simulink model "DAB_RA8P1_Final_Physical_MOSFET"  (R2024b)
settings: Solver=daessc  StartTime=0.0  StopTime=0.03  MaxStep=1e-8  RelTol=2e-3  AbsTol=1e-5
libraries: ee_lib x118, fl_lib x18, nesl_utility x15
(part 6 of 6)

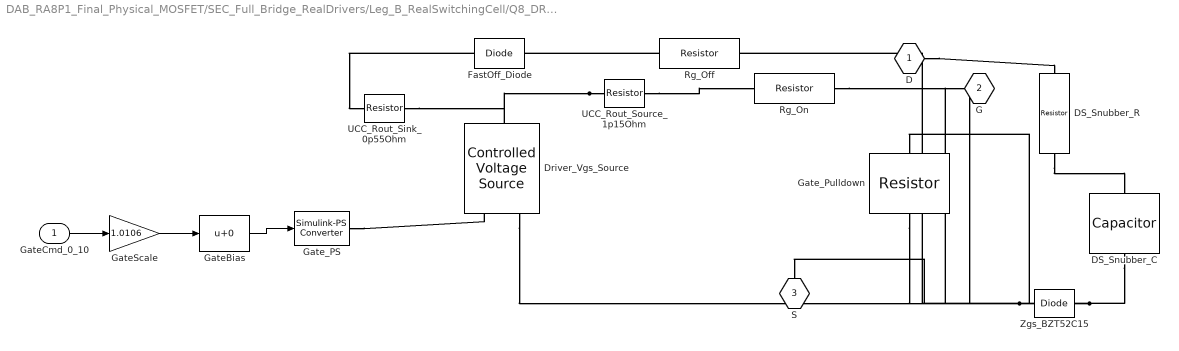
== system DAB_RA8P1_Final_Physical_MOSFET/SEC_Full_Bridge_RealDrivers/Leg_B_RealSwitchingCell/Q8_DRV_EQ ==
  GateCmd_0_10 : Inport
  DS_Snubber_C : ee_lib/Passive/Capacitor  cap_option=ee.enum.passive.capacitor.capOption.const  c=470 pF  Cvec=[1e-05, 1e-06] F  Vvec=[0, 10] V  CV_table_symmetry=ee.enum.passive.capacitor.tableSymmetry.yes  f_vec=[1, 10] kHz  DFext_vec=[.8, 1.2]  enable_C_tol=ee.enum.toleranceApplication.none  averaging_period=0 s  C_tol=5  tol_distribution=ee.enum.toleranceDistribution.uniform  nSigma=4  r=0.05 Ohm  g=0 1/Ohm  enable_operating_limits=ee.enum.enable.no  operating_limit_action=ee.enum.passive.reportOpLim.warn  max_working_voltage_range=[-25, 25] V  power_rating=1 W  maxTemperature=85 degC  thermalEnable=false  thermalMass=1 J/K  fault_action=simscape.enum.assert.action.none  t_fault=1 s  i_specify=off  i_priority=None  i=0 A  i_nominal_specify=off  i_nominal_value=1  i_nominal_unit=A  v_specify=off  v_priority=None  v=0 V  v_nominal_specify=off  v_nominal_value=1  v_nominal_unit=V  vc_specify=off  vc_priority=High  vc=0 V  vc_nominal_specify=off  vc_nominal_value=1  vc_nominal_unit=V  T_specify=off  T_priority=None  T=298.15 K  T_nominal_specify=off  T_nominal_value=1  T_nominal_unit=K
      settings: AttributesFormatString=Initial 470pF C0G snubber; DNP/tune after Vds measurement
  DS_Snubber_R : ee_lib/Passive/Resistor  R=10 Ohm  enable_R_tol=ee.enum.toleranceApplication.none  R_tol=5  tol_distribution=ee.enum.toleranceDistribution.uniform  nSigma=4  enable_operating_limits=ee.enum.enable.no  operating_limit_action=ee.enum.passive.reportOpLim.warn  power_rating=1 W  max_working_voltage=100 V  noise_mode=ee.enum.sources.noise.Disabled  Tdevice=25 degC  sample_time=1e-3 s  repeatability=ee.enum.ic.repeatability.notRepeatable  user_seed=0  auto_seed=1141249012  fault_action=simscape.enum.assert.action.none  t_fault=1 s  power_derating_T1=70 degC  power_derating_T2=155 degC  operating_temperature_range_vec=[-50, 150] degC  alpha=3.93e-3 1/K  Tmeas=25 degC  thermal_mass=100 J/K  temperature_specify=off  temperature_priority=High  temperature=298.15 K  temperature_nominal_specify=off  temperature_nominal_value=1  temperature_nominal_unit=K
      settings: AttributesFormatString=Initial RC snubber value; tune by double-pulse measurement
  Driver_Vgs_Source : fl_lib/Electrical/Electrical Sources/Controlled Voltage Source
  FastOff_Diode : ee_lib/Semiconductors & Converters/Diode  ModelType=ee.enum.diode.modelType.pwl  TableType=ee.enum.diode.tableType.IfMat  IfMat=[.07, .12, .19, 1.75, 4.24, 7.32, 11.2; .16, .3, .72, 2.14, 5.02, 8.35, 13.12] A  VfMat=[.9, 1.15, 1.25, 1.5, 1.75, 2.17, 2.6, 2.85; .58, .68, .75, 1.1, 1.38, 1.77, 2.27, 2.7] V  TjVec=[25, 125] degC  VfVec=[.5, .7, .9, 1.3, 1.7, 2.1, 2.5] V  IfVec=[.1, .2, .5, 1, 2, 4, 7, 10] A  IrMat=[1e-06, 2e-06, 5e-06, 1e-05, 2.5e-05, 5e-05, .0001; 2e-06, 5e-06, 1e-05, 4e-05, 8e-05, .0002, .0005] A  VrMat=[10, 100, 200, 250, 300, 325, 350; 10, 70, 160, 220, 270, 300, 320] V  VrVec=[10, 20, 40, 50, 70, 80, 100] V  IrVec=[1e-06, 2e-06, 5e-06, 1e-05, 2e-05, 5e-05, .0001] A  Vf=0.30 V  Ron=0.19 Ohm  Goff=1e-8 S  prmExp=ee.enum.diode.expParam.useTwo  I12=[.0137, .545] A  V12=[.6, .7] V  RS=0 Ohm  Tmeas=298.15 K  IS=1e-12 A  ec=1  I1=0.0137 A  V1=0.6 V  N_series=1  N_parallel=1  ZenerEnable=false  Rz=0.3 Ohm  BV=40 V  C_param=ee.enum.diode.capParam.fixed  CJ=0 pF  CJ0=5 pF  Vvec=[.1, 10, 100] V  Cvec=[3.5, 1, .4] pF  VJ=1 V  Mgrad=0.5  FC=0.5  Q_param=ee.enum.diode.recoveryParam.off  iRM=-7.15 A  iF=4 A  didt=-750 A/us  trr_factor=3  trr=115 ns  Qrr=150 nA*s  Vr=-600 V  Ls=150 nH  Erec=0.03 J  TT=50 ns  tau=100 ns  T_param=ee.enum.diode.temperatureParam.off  Tdevice=298.15 K  I1_T2=0.245 A  V1_T2=0.5 V  IS_T2=1.25e-7 A  Tmeas2=125 degC  XTI_param=ee.enum.diode.xtiParam.pn  XTI=3  EG_param=ee.enum.diode.egapParam.material_si  EG=1.11 eV  dBVdT=0 V/K  fault_action=simscape.enum.assert.action.none  t_fault=inf s  enable_fault_input=simscape.enum.onoff.off  i_specify=off  i_priority=None  i=0 A  i_nominal_specify=off  i_nominal_value=1  i_nominal_unit=A  v_specify=off  v_priority=None  v=0 V  v_nominal_specify=off  v_nominal_value=1  v_nominal_unit=V  v_capacitor_specify=off  v_capacitor_priority=None  v_capacitor=0 V  v_capacitor_nominal_specify=off  v_capacitor_nominal_value=1  v_capacitor_nominal_unit=V  Qj_specify=off  Qj_priority=High  Qj=0 C  Qj_nominal_specify=off  Qj_nominal_value=1  Qj_nominal_unit=C  i_diode_specify=off  i_diode_priority=None  i_diode=0 A  i_diode_nominal_specify=off  i_diode_nominal_value=1  i_diode_nominal_unit=A  v_diode_specify=off  v_diode_priority=None  v_diode=0 V  v_diode_nominal_specify=off  v_diode_nominal_value=1  v_diode_nominal_unit=V  i_capacitor_specify=off  i_capacitor_priority=None  i_capacitor=0 A  i_capacitor_nominal_specify=off  i_capacitor_nominal_value=1  i_capacitor_nominal_unit=A  power_dissipated_specify=off  power_dissipated_priority=None  power_dissipated=0 W  power_dissipated_nominal_specify=off  power_dissipated_nominal_value=1  power_dissipated_nominal_unit=W  fidelity_level=ee.enum.diode.fidelity.includeChargeDyn  rec_loss_model=ee.enum.diode.reverseRecoveryModel.fixed  ErecVal=0 J  scaleWithIandV=true  ErecMat=zeros(2, 3) J  TjrecVec=[298.15, 398.15] K  IfrecVec=[.1, 1, 10] A  IrecVal=10 A  VrecVal=10 V  tFilter=1 / 1000 / 100 s  thermal_network_parameterization=ee.enum.thermalNetworkTopology.junctionCase  Rth=[0, 10] K/W  Rth_Cauer=[1, 3, 10] K/W  Rth_Foster=[.08, .14, .22, .16] K/W  thermal_mass_parameterization=ee.enum.thermalNetwork.timeconstant  thermal_mass=[0, 1] J/K  thermal_mass_Cauer=[.1, .3, 1] J/K  thermal_mass_Foster=[.001, .005, .05, .5] J/K  thermal_time_constant=[0, 10] s  thermal_time_constant_Cauer=[1, 3, 10] s  thermal_time_constant_Foster=[7e-05, .0007, .01, .08] s  thermal_mass_initial_temperatures=[25, 25] degC  thermal_mass_initial_temperatures_Cauer=[25, 25, 25] degC  junction_thermal_mass=0.01 J/K  Tvec_initial_Foster=[25, 25, 25, 25] degC  no_thermal_network=0  junction_temperature_specify=off  junction_temperature_priority=None  junction_temperature=25 degC  junction_temperature_nominal_specify=off  junction_temperature_nominal_value=1  junction_temperature_nominal_unit=degC
  GateBias : Bias  SaturateOnIntegerOverflow=off
  GateScale : Gain  Gain=1.0106
  Gate_PS : nesl_utility/Simulink-PS Converter  PhysicalDomain=network_engine_domain  SubClassName=ps_input  LeftPortType=input  RightPortType=output  PseudoPeriodic=off  Frequencies=[]  NoiseDistribution=none  NoiseParameters=[]  Unit=V  AffineConversion=off  FilteringAndDerivatives=provide  SimscapeFilterOrder=1  InputFilterTimeConstant=0.001  UdotUserProvided=0
  Gate_Pulldown : ee_lib/Passive/Resistor  R=10000 Ohm  enable_R_tol=ee.enum.toleranceApplication.none  R_tol=5  tol_distribution=ee.enum.toleranceDistribution.uniform  nSigma=4  enable_operating_limits=ee.enum.enable.no  operating_limit_action=ee.enum.passive.reportOpLim.warn  power_rating=1 W  max_working_voltage=100 V  noise_mode=ee.enum.sources.noise.Disabled  Tdevice=25 degC  sample_time=1e-3 s  repeatability=ee.enum.ic.repeatability.notRepeatable  user_seed=0  auto_seed=1157818018  fault_action=simscape.enum.assert.action.none  t_fault=1 s  power_derating_T1=70 degC  power_derating_T2=155 degC  operating_temperature_range_vec=[-50, 150] degC  alpha=3.93e-3 1/K  Tmeas=25 degC  thermal_mass=100 J/K  temperature_specify=off  temperature_priority=High  temperature=298.15 K  temperature_nominal_specify=off  temperature_nominal_value=1  temperature_nominal_unit=K
  Rg_Off : ee_lib/Passive/Resistor  R=2.2 Ohm  enable_R_tol=ee.enum.toleranceApplication.none  R_tol=5  tol_distribution=ee.enum.toleranceDistribution.uniform  nSigma=4  enable_operating_limits=ee.enum.enable.no  operating_limit_action=ee.enum.passive.reportOpLim.warn  power_rating=1 W  max_working_voltage=100 V  noise_mode=ee.enum.sources.noise.Disabled  Tdevice=25 degC  sample_time=1e-3 s  repeatability=ee.enum.ic.repeatability.notRepeatable  user_seed=0  auto_seed=4137157194  fault_action=simscape.enum.assert.action.none  t_fault=1 s  power_derating_T1=70 degC  power_derating_T2=155 degC  operating_temperature_range_vec=[-50, 150] degC  alpha=3.93e-3 1/K  Tmeas=25 degC  thermal_mass=100 J/K  temperature_specify=off  temperature_priority=High  temperature=298.15 K  temperature_nominal_specify=off  temperature_nominal_value=1  temperature_nominal_unit=K
  Rg_On : ee_lib/Passive/Resistor  R=4.7 Ohm  enable_R_tol=ee.enum.toleranceApplication.none  R_tol=5  tol_distribution=ee.enum.toleranceDistribution.uniform  nSigma=4  enable_operating_limits=ee.enum.enable.no  operating_limit_action=ee.enum.passive.reportOpLim.warn  power_rating=1 W  max_working_voltage=100 V  noise_mode=ee.enum.sources.noise.Disabled  Tdevice=25 degC  sample_time=1e-3 s  repeatability=ee.enum.ic.repeatability.notRepeatable  user_seed=0  auto_seed=2368526529  fault_action=simscape.enum.assert.action.none  t_fault=1 s  power_derating_T1=70 degC  power_derating_T2=155 degC  operating_temperature_range_vec=[-50, 150] degC  alpha=3.93e-3 1/K  Tmeas=25 degC  thermal_mass=100 J/K  temperature_specify=off  temperature_priority=High  temperature=298.15 K  temperature_nominal_specify=off  temperature_nominal_value=1  temperature_nominal_unit=K
  UCC_Rout_Sink_0p55Ohm : ee_lib/Passive/Resistor  R=0.55 Ohm  enable_R_tol=ee.enum.toleranceApplication.none  R_tol=5  tol_distribution=ee.enum.toleranceDistribution.uniform  nSigma=4  enable_operating_limits=ee.enum.enable.no  operating_limit_action=ee.enum.passive.reportOpLim.warn  power_rating=1 W  max_working_voltage=100 V  noise_mode=ee.enum.sources.noise.Disabled  Tdevice=25 degC  sample_time=1e-3 s  repeatability=ee.enum.ic.repeatability.notRepeatable  user_seed=0  auto_seed=609397185  fault_action=simscape.enum.assert.action.none  t_fault=1 s  power_derating_T1=70 degC  power_derating_T2=155 degC  operating_temperature_range_vec=[-50, 150] degC  alpha=3.93e-3 1/K  Tmeas=25 degC  thermal_mass=100 J/K  temperature_specify=off  temperature_priority=High  temperature=298.15 K  temperature_nominal_specify=off  temperature_nominal_value=1  temperature_nominal_unit=K
  UCC_Rout_Source_1p15Ohm : ee_lib/Passive/Resistor  R=1.15 Ohm  enable_R_tol=ee.enum.toleranceApplication.none  R_tol=5  tol_distribution=ee.enum.toleranceDistribution.uniform  nSigma=4  enable_operating_limits=ee.enum.enable.no  operating_limit_action=ee.enum.passive.reportOpLim.warn  power_rating=1 W  max_working_voltage=100 V  noise_mode=ee.enum.sources.noise.Disabled  Tdevice=25 degC  sample_time=1e-3 s  repeatability=ee.enum.ic.repeatability.notRepeatable  user_seed=0  auto_seed=3437178441  fault_action=simscape.enum.assert.action.none  t_fault=1 s  power_derating_T1=70 degC  power_derating_T2=155 degC  operating_temperature_range_vec=[-50, 150] degC  alpha=3.93e-3 1/K  Tmeas=25 degC  thermal_mass=100 J/K  temperature_specify=off  temperature_priority=High  temperature=298.15 K  temperature_nominal_specify=off  temperature_nominal_value=1  temperature_nominal_unit=K
  Zgs_BZT52C15 : ee_lib/Semiconductors & Converters/Diode  ModelType=ee.enum.diode.modelType.pwl  TableType=ee.enum.diode.tableType.IfMat  IfMat=[.07, .12, .19, 1.75, 4.24, 7.32, 11.2; .16, .3, .72, 2.14, 5.02, 8.35, 13.12] A  VfMat=[.9, 1.15, 1.25, 1.5, 1.75, 2.17, 2.6, 2.85; .58, .68, .75, 1.1, 1.38, 1.77, 2.27, 2.7] V  TjVec=[25, 125] degC  VfVec=[.5, .7, .9, 1.3, 1.7, 2.1, 2.5] V  IfVec=[.1, .2, .5, 1, 2, 4, 7, 10] A  IrMat=[1e-06, 2e-06, 5e-06, 1e-05, 2.5e-05, 5e-05, .0001; 2e-06, 5e-06, 1e-05, 4e-05, 8e-05, .0002, .0005] A  VrMat=[10, 100, 200, 250, 300, 325, 350; 10, 70, 160, 220, 270, 300, 320] V  VrVec=[10, 20, 40, 50, 70, 80, 100] V  IrVec=[1e-06, 2e-06, 5e-06, 1e-05, 2e-05, 5e-05, .0001] A  Vf=0.60 V  Ron=0.30 Ohm  Goff=1e-8 S  prmExp=ee.enum.diode.expParam.useTwo  I12=[.0137, .545] A  V12=[.6, .7] V  RS=0 Ohm  Tmeas=298.15 K  IS=1e-12 A  ec=1  I1=0.0137 A  V1=0.6 V  N_series=1  N_parallel=1  ZenerEnable=true  Rz=1 Ohm  BV=15 V  C_param=ee.enum.diode.capParam.fixed  CJ=0 pF  CJ0=5 pF  Vvec=[.1, 10, 100] V  Cvec=[3.5, 1, .4] pF  VJ=1 V  Mgrad=0.5  FC=0.5  Q_param=ee.enum.diode.recoveryParam.off  iRM=-7.15 A  iF=4 A  didt=-750 A/us  trr_factor=3  trr=115 ns  Qrr=150 nA*s  Vr=-600 V  Ls=150 nH  Erec=0.03 J  TT=50 ns  tau=100 ns  T_param=ee.enum.diode.temperatureParam.off  Tdevice=298.15 K  I1_T2=0.245 A  V1_T2=0.5 V  IS_T2=1.25e-7 A  Tmeas2=125 degC  XTI_param=ee.enum.diode.xtiParam.pn  XTI=3  EG_param=ee.enum.diode.egapParam.material_si  EG=1.11 eV  dBVdT=0 V/K  fault_action=simscape.enum.assert.action.none  t_fault=inf s  enable_fault_input=simscape.enum.onoff.off  i_specify=off  i_priority=None  i=0 A  i_nominal_specify=off  i_nominal_value=1  i_nominal_unit=A  v_specify=off  v_priority=None  v=0 V  v_nominal_specify=off  v_nominal_value=1  v_nominal_unit=V  v_capacitor_specify=off  v_capacitor_priority=None  v_capacitor=0 V  v_capacitor_nominal_specify=off  v_capacitor_nominal_value=1  v_capacitor_nominal_unit=V  Qj_specify=off  Qj_priority=High  Qj=0 C  Qj_nominal_specify=off  Qj_nominal_value=1  Qj_nominal_unit=C  i_diode_specify=off  i_diode_priority=None  i_diode=0 A  i_diode_nominal_specify=off  i_diode_nominal_value=1  i_diode_nominal_unit=A  v_diode_specify=off  v_diode_priority=None  v_diode=0 V  v_diode_nominal_specify=off  v_diode_nominal_value=1  v_diode_nominal_unit=V  i_capacitor_specify=off  i_capacitor_priority=None  i_capacitor=0 A  i_capacitor_nominal_specify=off  i_capacitor_nominal_value=1  i_capacitor_nominal_unit=A  power_dissipated_specify=off  power_dissipated_priority=None  power_dissipated=0 W  power_dissipated_nominal_specify=off  power_dissipated_nominal_value=1  power_dissipated_nominal_unit=W  fidelity_level=ee.enum.diode.fidelity.includeChargeDyn  rec_loss_model=ee.enum.diode.reverseRecoveryModel.fixed  ErecVal=0 J  scaleWithIandV=true  ErecMat=zeros(2, 3) J  TjrecVec=[298.15, 398.15] K  IfrecVec=[.1, 1, 10] A  IrecVal=10 A  VrecVal=10 V  tFilter=1 / 1000 / 100 s  thermal_network_parameterization=ee.enum.thermalNetworkTopology.junctionCase  Rth=[0, 10] K/W  Rth_Cauer=[1, 3, 10] K/W  Rth_Foster=[.08, .14, .22, .16] K/W  thermal_mass_parameterization=ee.enum.thermalNetwork.timeconstant  thermal_mass=[0, 1] J/K  thermal_mass_Cauer=[.1, .3, 1] J/K  thermal_mass_Foster=[.001, .005, .05, .5] J/K  thermal_time_constant=[0, 10] s  thermal_time_constant_Cauer=[1, 3, 10] s  thermal_time_constant_Foster=[7e-05, .0007, .01, .08] s  thermal_mass_initial_temperatures=[25, 25] degC  thermal_mass_initial_temperatures_Cauer=[25, 25, 25] degC  junction_thermal_mass=0.01 J/K  Tvec_initial_Foster=[25, 25, 25, 25] degC  no_thermal_network=0  junction_temperature_specify=off  junction_temperature_priority=None  junction_temperature=25 degC  junction_temperature_nominal_specify=off  junction_temperature_nominal_value=1  junction_temperature_nominal_unit=degC
  D : PMIOPort  Side=Right
  G : PMIOPort  Port=2  Side=Right
  S : PMIOPort  Port=3  Side=Right
  wires:
  GateCmd_0_10/1 -> GateScale/1
  GateScale/1 -> GateBias/1
  GateBias/1 -> Gate_PS/1
  connections:
  Gate_PS/RConn1 -- Driver_Vgs_Source/RConn1
  Rg_On/RConn1 -- Zgs_BZT52C15/RConn1 -- Rg_Off/LConn1 -- G/RConn1 -- Gate_Pulldown/LConn1
  Rg_Off/RConn1 -- FastOff_Diode/LConn1
  Gate_Pulldown/RConn1 -- Driver_Vgs_Source/RConn2 -- Zgs_BZT52C15/LConn1 -- S/RConn1 -- DS_Snubber_C/RConn1
  D/RConn1 -- DS_Snubber_R/LConn1
  DS_Snubber_R/RConn1 -- DS_Snubber_C/LConn1
  UCC_Rout_Source_1p15Ohm/LConn1 -- Driver_Vgs_Source/LConn1 -- UCC_Rout_Sink_0p55Ohm/RConn1
  UCC_Rout_Source_1p15Ohm/RConn1 -- Rg_On/LConn1
  FastOff_Diode/RConn1 -- UCC_Rout_Sink_0p55Ohm/LConn1

== matlab function DAB_RA8P1_Final_Physical_MOSFET/RA8P1_Realtime_Voltage_PI ==
  settings: updateMethod=DISCRETE  sampleTime=1e-8
  data: t input; g1 output; Vout input; VrefCmd input; Vin input; Iout input; Ipri input; Isec input; g2 output; g3 output; g4 output; g5 output; g6 output; g7 output; g8 output; PhaseUs output; RunReq input; RawFaultN input
function [g1,g2,g3,g4,g5,g6,g7,g8,PhaseUs] = f(t,Vout,VrefCmd,Vin,Iout,Ipri,Isec,RunReq,RawFaultN)
%#codegen
% Cold start: alternating primary three-level pulses, secondary gates off.
% NORMAL mode starts only after 20 consecutive voltage-domain samples.
% RawFaultN is the modeled hardware FAULT_LATCH_N signal.
persistent trim prevErr lastTick vFilt vinFilt iFilt permitCount normalEnabled startupEnabled startupCycle startupPulseAllowed startupPolarity normalRamp iPriPeakHold iSecPeakHold startupPulseCmd startupIpriCyclePeak startupIsecCyclePeak epsTrim epsQuantAcc epsPhaseCmd
if isempty(trim)
    trim = 0;
    prevErr = 0;
    lastTick = -1;
    vFilt = 0;
    vinFilt = 24;
    iFilt = 0;
    permitCount = uint16(0);
    normalEnabled = false;
    startupEnabled = false;
    startupCycle = -1;
    startupPulseAllowed = false;
    startupPolarity = false;
    normalRamp = 0;
    iPriPeakHold = 0;
    iSecPeakHold = 0;
    startupPulseCmd = 100e-9;
    startupIpriCyclePeak = 0;
    startupIsecCyclePeak = 0;
    epsTrim = 0;
    epsQuantAcc = 0;
    epsPhaseCmd = 0.30e-6;
end
fs = 300e3;
T = 1/fs;
deadTime = 120e-9;
TsCtrl = 10e-6;
tick = floor(t/TsCtrl);
Vref = min(max(VrefCmd,36),48);
rawVoltageOk = Vin >= 18 && Vin <= 28 && Vout >= -0.5 && Vout < 50;
faultOk = RunReq > 0.5 && RawFaultN > 0.5 && rawVoltageOk;
iPriPeakHold = max(iPriPeakHold,abs(Ipri));
iSecPeakHold = max(iSecPeakHold,abs(Isec));
startupIpriCyclePeak = max(startupIpriCyclePeak,abs(Ipri));
startupIsecCyclePeak = max(startupIsecCyclePeak,abs(Isec));
if tick ~= lastTick
    if lastTick < 0
        vFilt = Vout;
        vinFilt = Vin;
        iFilt = abs(Iout);
    else
        vFilt = vFilt + 0.40*(Vout - vFilt);
        vinFilt = vinFilt + 0.10*(Vin - vinFilt);
        iFilt = iFilt + 0.22*(abs(Iout) - iFilt);
    end
    ratioMismatch = abs(Vout - 2*Vin);
    entryRatioOk = (Vout < 2*Vin && ratioMismatch <= 7.0) || ...
        (Vout >= 2*Vin && ratioMismatch <= 12.5);
    holdRatioOk = (Vout < 2*Vin && ratioMismatch < 10.0) || ...
        (Vout >= 2*Vin && ratioMismatch < 13.5);
    startupOk = faultOk && vinFilt >= 18 && vinFilt <= 28 && ...
        vFilt >= -0.5 && vFilt < 50;
    entryOk = faultOk && vinFilt >= 18 && vinFilt <= 28 && ...
        vFilt >= 36 && vFilt <= 48 && entryRatioOk;
    holdOk = faultOk && vinFilt >= 18 && vinFilt <= 28 && ...
        vFilt >= 36 && vFilt <= 49.0 && holdRatioOk;
    if normalEnabled
        if ~holdOk
            normalEnabled = false;
            startupEnabled = startupOk;
            startupPulseCmd = startup_pulse_width(Vout,Vin);
            startupCycle = -1;
            startupPolarity = false;
            permitCount = uint16(0);
            trim = 0;
            normalRamp = 0;
        end
    else
        if ~startupOk
            startupEnabled = false;
            permitCount = uint16(0);
        elseif entryOk
            startupEnabled = false;
            if permitCount < uint16(20)
                permitCount = permitCount + uint16(1);
            end
        else
            if ~startupEnabled
                startupPulseCmd = startup_pulse_width(Vout,Vin);
                startupCycle = -1;
                startupPolarity = false;
                startupIpriCyclePeak = 0;
                startupIsecCyclePeak = 0;
            end
            startupEnabled = true;
            permitCount = uint16(0);
        end
        if permitCount >= uint16(20)
            normalEnabled = true;
            startupEnabled = false;
            normalRamp = 0;
            trim = 0;
            prevErr = Vref - vFilt;
        end
    end
    if normalEnabled
        normalIpriLow = min(48,36 + 1.2*iFilt);
        normalIsecLow = min(24,18 + 0.6*iFilt);
        if iPriPeakHold < normalIpriLow && iSecPeakHold < normalIsecLow
            normalRamp = min(1,normalRamp + 0.005);
        elseif iPriPeakHold >= normalIpriLow + 4 || iSecPeakHold >= normalIsecLow + 2
            normalRamp = max(0,normalRamp - 0.05);
        end
        err = Vref - vFilt;
        dErr = err - prevErr;
        trim = 0.965*trim + 0.0102e-6*err + 0.0033e-6*dErr;
        trimLimit = 0.100e-6;
        if iFilt < 0.70
            trimLimit = 0.016e-6;
        end
        trim = min(max(trim, -trimLimit), trimLimit);
        prevErr = err;
        if iFilt >= 4
            epsTrim = min(max(epsTrim + 0.5e-9*err,-25e-9),25e-9);
            epsDesired = min(max(0.295e-6 + epsTrim + 0.20e-6*err,0.28e-6),0.32e-6);
            epsLow = floor(epsDesired/10e-9)*10e-9;
            epsQuantAcc = epsQuantAcc + (epsDesired-epsLow)/10e-9;
            epsPhaseCmd = epsLow;
            if epsQuantAcc >= 1
                epsPhaseCmd = epsLow + 10e-9;
                epsQuantAcc = epsQuantAcc - 1;
            end
        else
            epsTrim = 0;
            epsQuantAcc = 0;
            epsPhaseCmd = 0.30e-6;
        end
    else
        trim = 0;
        normalRamp = 0;
        epsTrim = 0;
        epsQuantAcc = 0;
        epsPhaseCmd = 0.30e-6;
    end
    iPriPeakHold = abs(Ipri);
    iSecPeakHold = abs(Isec);
    lastTick = tick;
end
if normalEnabled && faultOk && iFilt >= 4
    % Physical-model EPS PI around the measured 0.295 us balance point.
    % epsPhaseCmd uses 10 ns timer quantization with pulse-density dither.
    if iPriPeakHold < 50 && iSecPeakHold < 28
        inner = 0.20e-6;
        phase = epsPhaseCmd;
        [a,an] = halfbridge(t,T,deadTime);
        [b,bn] = halfbridge(t+T/2-inner,T,deadTime);
        [c,cn] = halfbridge(t-phase,T,deadTime);
        [d,dn] = halfbridge(t-phase+T/2,T,deadTime);
        g1 = 10*a;  g2 = 10*an;
        g3 = 10*b;  g4 = 10*bn;
        g5 = 10*c;  g6 = 10*cn;
        g7 = 10*d;  g8 = 10*dn;
        PhaseUs = phase*1e6;
    else
        g1 = 0; g2 = 0; g3 = 0; g4 = 0;
        g5 = 0; g6 = 0; g7 = 0; g8 = 0;
        PhaseUs = 0;
    end
elseif normalEnabled && faultOk
    phase = normalRamp*(base_phase(Vref, vinFilt, iFilt) + trim);
    phase = min(max(phase, -0.55e-6), 0.46e-6);
    [a,an] = halfbridge(t,T,deadTime);
    [b,bn] = halfbridge(t+T/2,T,deadTime);
    [c,cn] = halfbridge(t-phase,T,deadTime);
    [d,dn] = halfbridge(t-phase+T/2,T,deadTime);
    g1 = 10*a;  g2 = 10*an;
    g3 = 10*b;  g4 = 10*bn;
    g5 = 10*c;  g6 = 10*cn;
    g7 = 10*d;  g8 = 10*dn;
    PhaseUs = phase*1e6;
elseif startupEnabled && faultOk
    startupSlotPeriod = T/2;
    cycle = floor(t/startupSlotPeriod);
    if cycle ~= startupCycle
        if startupCycle >= 0
            adaptDeltaV = max(Vin - 0.5*Vout,2);
            pulseStepUp = 5e-9 + 15e-9*min(max((10-adaptDeltaV)/6,0),1);
            if startupIpriCyclePeak < 28 && startupIsecCyclePeak < 14
                startupPulseCmd = startupPulseCmd + pulseStepUp;
            elseif startupIpriCyclePeak > 31 || startupIsecCyclePeak > 16
                startupPulseCmd = startupPulseCmd - 40e-9;
            end
        end
        startupPulseCmd = max(startupPulseCmd,startup_pulse_width(Vout,Vin));
        startupPulseCmd = min(max(startupPulseCmd,100e-9),1.3e-6);
        startupDeltaV = max(Vin - 0.5*Vout,2);
        if startupDeltaV >= 12
            highDeltaCap = 26*0.1e-6/startupDeltaV + 35e-9;
            startupPulseCmd = min(startupPulseCmd,highDeltaCap);
        end
        if Vout < 15
            % 24A volt-second cap using 0.4uH secondary leakage / 4.
            lowVoltageCap = 24*0.1e-6/startupDeltaV;
            lowVoltageCap = min(max(lowVoltageCap,100e-9),185e-9);
            startupPulseCmd = min(startupPulseCmd,lowVoltageCap);
        end
        startupPulseAllowed = abs(Ipri) < 3 && abs(Isec) < 3 && ...
            Vout < Vref - 0.05;
        if startupPulseAllowed
            startupPolarity = ~startupPolarity;
        end
        startupCycle = cycle;
        startupIpriCyclePeak = abs(Ipri);
        startupIsecCyclePeak = abs(Isec);
    end
    if abs(Ipri) >= 35 || abs(Isec) >= 20
        startupPulseAllowed = false;
    end
    if startupPulseAllowed
        [p1,p2,p3,p4] = startup_bridge(t,startupSlotPeriod,deadTime,startupPulseCmd,startupPolarity);
        g1 = 10*p1; g2 = 10*p2; g3 = 10*p3; g4 = 10*p4;
    else
        g1 = 0; g2 = 0; g3 = 0; g4 = 0;
    end
    g5 = 0; g6 = 0; g7 = 0; g8 = 0;
    PhaseUs = startupPulseCmd*1e6*double(g1 > 0 || g2 > 0 || g3 > 0 || g4 > 0);
else
    g1 = 0; g2 = 0; g3 = 0; g4 = 0;
    g5 = 0; g6 = 0; g7 = 0; g8 = 0;
    PhaseUs = 0;
end
end

function pulseWidth = startup_pulse_width(Vout,Vin)
% Use the 0.4uH secondary-referred minimum leakage (0.1uH primary).
deltaV = max(Vin - 0.5*Vout,2);
pulseWidth = 30*0.1e-6/deltaV;
delayComp = 100e-9*min(max((15-deltaV)/10,0),1);
pulseWidth = pulseWidth + delayComp;
pulseWidth = min(max(pulseWidth,100e-9),900e-9);
end

function [q1,q2,q3,q4] = startup_bridge(t,T,deadTime,pulseWidth,polarity)
x = mod(t,T);
active = double(x >= deadTime && x < deadTime + pulseWidth);
freewheel = double(x >= deadTime + pulseWidth + deadTime);
lowAfterBoundary = double(x >= deadTime);
if polarity
    q1 = active; q2 = freewheel; q3 = 0; q4 = lowAfterBoundary;
else
    q1 = 0; q2 = lowAfterBoundary; q3 = active; q4 = freewheel;
end
end

function phase = base_phase(Vref,Vin,Iout)
buckDelta = Vin - 0.5*Vref;
if buckDelta > 0.6
    light = max(0, 1.7 - Iout);
    lowBuckTrim = 0.0096*exp(-((buckDelta - 2.0)/2.0)^2) + 0.0040*exp(-((buckDelta - 4.0)/1.2)^2);
    lightBuckTrim = 0.0085*exp(-((Iout - 0.52)/0.22)^2)*min(max((buckDelta - 2.0)/4.0, 0), 1);
    midBuckGain = 0.012 + 0.012*min(max((buckDelta - 2.0)/4.0, 0), 1);
    midBuckLoadTrim = midBuckGain*exp(-((Iout - 1.22)/0.42)^2);
    lowBuckMidRelief = 0.0076*exp(-((Iout - 1.10)/0.30)^2)*exp(-((buckDelta - 2.0)/0.90)^2);
    highBuckLoad = max(Iout - 3.2, 0);
    highBuckReliefRaw = 0.0038*highBuckLoad^2 + 0.0050*max(Iout - 10.0, 0)^2 + 0.0340*max(Iout - 11.5, 0)^2;
    highBuckRelief = min(highBuckReliefRaw, 0.594);
    phaseUs = -0.229 - 0.0165*buckDelta - 0.0110*min(Iout,3.2) - 0.020*light - lowBuckTrim - lightBuckTrim - midBuckLoadTrim + lowBuckMidRelief + highBuckRelief;
else
    highBoostLoad = max(Iout - 3.0, 0);
    highBoostBackoff = 0.128*(1 - exp(-highBoostLoad/1.6)) + 0.02925*max(Iout - 7.0, 0);
    phaseUs = -0.028 + 0.112*min(Iout,2.3) + 0.038*max(Iout-1.4,0) - highBoostBackoff;
end
if buckDelta > 0.6
    phaseUs = phaseUs + 0.095*exp(-((Iout - 13.0)/3.0)^2)*exp(-((buckDelta - 6.0)/1.4)^2);
else
    phaseUs = phaseUs + 0.010*(1 - exp(-max(Iout - 7.0, 0)/2.0));
    phaseUs = phaseUs + 0.020*exp(-(buckDelta/0.75)^2)*exp(-((Iout - 2.1)/1.0)^2);
end
phase = min(max(phaseUs*1e-6, -0.55e-6), 0.46e-6);
end

function [hi,lo] = halfbridge(t,T,deadTime)
x = mod(t,T);
halfDead = deadTime/2;
hi = double(x >= halfDead && x < T/2 - halfDead);
lo = double(x >= T/2 + halfDead && x < T - halfDead);
end

== matlab function DAB_RA8P1_Final_Physical_MOSFET/Power_Efficiency_Calc ==
  data: Vin input; IinAbs output; Iin input; Vout input; Iout input; IoutAbs output; Pin output; Pout output; Efficiency output
function [IinAbs,IoutAbs,Pin,Pout,Efficiency] = f(Vin,Iin,Vout,Iout)
%#codegen
IinAbs = Iin;
IoutAbs = Iout;
Pin = Vin * IinAbs;
Pout = Vout * Iout;
if Pin > 0.2
    Efficiency = min(max(100 * max(Pout,0) / Pin, 0), 100);
else
    Efficiency = 0;
end
end

== matlab function DAB_RA8P1_Final_Physical_MOSFET/Hardware_Fault_Latch_N ==
  settings: updateMethod=DISCRETE  sampleTime=1e-8
  data: RawFaultN input; FaultLatchN output; RunReq input
function FaultLatchN = f(RawFaultN,RunReq)
%#codegen
% Simulates U_LATCH. Real PCB reset remains a separate MCU pulse.
persistent faultLatched
if isempty(faultLatched)
    faultLatched = false;
end
if RawFaultN <= 0.5
    faultLatched = true;
elseif RunReq <= 0.5
    faultLatched = false;
end
FaultLatchN = double(~faultLatched);
end
